simulink model "three_phase_bridge_three_level_ttype_igbt_simple_2th"  (R2026b)
settings: Solver=VariableStepAuto
undefined symbols (not defined in the file): param
libraries: fl_lib x192, nesl_utility x120, igbt_simple_2th_lib x12
(part 1 of 4)
settings Model: Creator=pwr-control  LastModifiedBy=d.bagnara

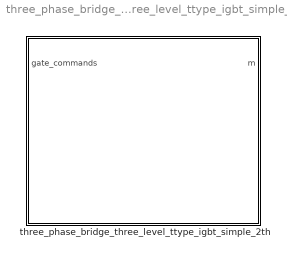
== system three_phase_bridge_three_level_ttype_igbt_simple_2th ==
  three_phase_bridge_three_level_ttype_igbt_simple_2th : Subsystem  mask(three_phase_bridge_three_level_ttype_igbt_simple_2th){vce_sat_m=param.afe.igbt.Vce_sat, rce_on_m=param.afe.igbt.Rce_on*1000, v_gamma_m=param.afe.igbt.Vdon_diode, rd_on_m=param.afe.igbt.Rdon_diode*1e3, Gce_off_m=1e-6, Vth_gate_m=param.afe.igbt.Vth, Vth_gate_hyst_m=0.85, Eon_m=param.afe.igbt.Eon*1000, Eoff_m=param.afe.igbt.Eoff*1000, Err_m=param.afe.igbt.Erec*1000, Ic_ref_m=param.afe.igbt.Ion_sw_losses, Vdc_ref_m=param.afe.igbt.Voff_sw_losses, Vblock_Errf_m=50, time_constant_edge_m=param.glb_time.tc*1e6, time_constant_ploss_m=param.glb_time.tPWM_AFE*5*1e6, Csnubber_m=12e-12, Rsnubber_m=2200, rth_switch_JH_m=param.afe.igbt.Rth_switch_JH, rth_switch_HA_m=param.thermal.Rth_switch_HA, rth_diode_JH_m=param.thermal.Rth_diode_HA, rth_diode_HA_m=param.thermal.Rth_diode_HA, JunctionTermalMass_m=param.afe.igbt.JunctionTermalMass, Tambient_m=param.thermal.Tambient, mass_heatsink_m=param.thermal.weight, specific_heat_m=param.thermal.cp_al}
      mask prompts: vce_sat_m "Collector-emitter on-state voltage (knee) [V]"; rce_on_m "IGBT on-state series resistance (slope) [mOhm]"; v_gamma_m "Diode forward voltage (knee) [V]"; rd_on_m "Diode series resistance (slope) [mOhm]"; Gce_off_m "Off-state conductance [1/Ohm]"; Vth_gate_m "Gate-emitter threshold voltage [V]"; Vth_gate_hyst_m "Half hysteresis band for the switching events [V]"; Eon_m "Turn-on energy at Ic_ref, Vdc_ref [mJ]"; Eoff_m "Turn-off energy at Ic_ref, Vdc_ref [mJ]"; Err_m "Reverse recovery energy at Ic_ref, Vdc_ref [mJ]"; Ic_ref_m "Reference current of the energies [A]"; Vdc_ref_m "Reference voltage of the energies [V]"; Vblock_Errf_m "Blocking detection level for the Err event [V]"; time_constant_edge_m "Sample&hold time constant (<< on-time) [us]"; time_constant_ploss_m "Loss averaging time constant (2-5 x Tsw) [us]"; Csnubber_m "RC snubber capacitance [F]"; Rsnubber_m "RC snubber resistance [Ohm]"; rth_switch_JH_m "Thermal resistance junction-heatsink, transistor die [K/W]"; rth_switch_HA_m "Thermal resistance heatsink-ambient, transistor die [K/W]"; rth_diode_JH_m "Thermal resistance junction-heatsink, diode die [K/W]"; rth_diode_HA_m "Thermal resistance heatsink-ambient, diode die [K/W]"; JunctionTermalMass_m "Junction thermal mass of each die [J/K]"; Tambient_m "Ambient temperature [degC]"; mass_heatsink_m "Heatsink mass seen by each die [kg]"; specific_heat_m "Specific heat of the heatsink [J/(K kg)]"
      mask help: Three-phase bridge, three-level T-type, igbt_simple_2th devices. IGBT cells built on igbt_simple_2th (library/foundation/semiconductors): knee + slope conduction, switching energies scaled from one datasheet point, separate thermal ports for the IGBT and the free-wheeling diode. Each die drives its own junction thermal mass -> Rth JH -> heatsink mass -> Rth HA -> ambient temperature source. Gate command in volts (modulators: +15/-10 V). Bus m per device k: igbt_current, igbt_voltage, igbt_ploss, igbt_JH_temp, igbt_HA_temp, diode_current, diode_ploss, diode_JH_temp, diode_HA_temp (temperatures are differences in K). Default data: Infineon FF450R17ME4 at 125 degC. Ports: gate_commands (bus from the three-level PWM modulators of masked_models/modulators), m (measurement bus), left dc terminals udc(+) / np / udc(-), right ac terminals u / v / w. Device numbering: see three_phase_bridge/README.md.
      mask Help: web('https://github.com/pwr-control/library/blob/dev/library/masked_models/semiconductors_bridges/three_phase_bridge/README.md', '-browser')
      mask DialogControl ParameterGroupVar Prompt: Conduction
      mask DialogControl ParameterGroupVar1 Prompt: Gate
      mask DialogControl ParameterGroupVar2 Prompt: Switching energies
      mask DialogControl ParameterGroupVar3 Prompt: Numerics and snubber
      mask DialogControl ParameterGroupVar4 Prompt: Thermal network
      mask Display:
      | disp(sprintf('three-phase bridge\nT-type 3 levels\nigbt_simple_2th'))
      | port_label('input', 1, 'gate_commands')
      | port_label('output', 1, 'm')
      | port_label('LConn', 1, 'udc(+)')
      | port_label('LConn', 2, 'np')
      | port_label('LConn', 3, 'udc(-)')
      | port_label('RConn', 1, 'u')
      | port_label('RConn', 2, 'v')
      | port_label('RConn', 3, 'w')

== system three_phase_bridge_three_level_ttype_igbt_simple_2th/three_phase_bridge_three_level_ttype_igbt_simple_2th ==
  gate_commands : Inport
  Bus Creator : BusCreator  Inputs=108
  Bus Selector : BusSelector  OutputSignals=gate_cmds_phu.cmd_gate_Q1,gate_cmds_phu.cmd_gate_Q2,gate_cmds_phu.cmd_gate_Q3,gate_cmds_phu.cmd_gate_Q4,gate_cmds_phv.cmd_gate_Q1,gate_cmds_phv.cmd_gate_Q2,gate_cmds_phv.cmd_gate_Q3,gate_cmds_phv.cmd_gate_Q4,gate_cmds_phw.cmd_gate_Q1,gate_cmds_phw.cmd_gate_Q2,gate_cmds_phw.cmd_gate_Q3,gate_cmds_phw.cmd_gate_Q4
  Q1 : Subsystem
  Q10 : Subsystem
  Q11 : Subsystem
  Q12 : Subsystem
  Q2 : Subsystem
  Q3 : Subsystem
  Q4 : Subsystem
  Q5 : Subsystem
  Q6 : Subsystem
  Q7 : Subsystem
  Q8 : Subsystem
  Q9 : Subsystem
  udc(+) : PMIOPort  Side=Left
  np : PMIOPort  Port=2  Side=Left
  udc(-) : PMIOPort  Port=3  Side=Left
  u : PMIOPort  Port=4  Side=Right
  v : PMIOPort  Port=5  Side=Right
  w : PMIOPort  Port=6  Side=Right
  m : Outport
  wires:
  gate_commands/1 -> Bus Selector/1
  Q9/3(p_t) -> Bus Creator/75  "igbt_ploss_Q9"
  Q6/2(v) -> Bus Creator/47  "igbt_voltage_Q6"
  Bus Selector/1 -> Q1/1(g)  "<cmd_gate_Q1>"
  Bus Selector/3 -> Q3/1(g)  "<cmd_gate_Q3>"
  Q3/7(p_d) -> Bus Creator/25  "diode_ploss_Q3"
  Bus Selector/5 -> Q5/1(g)  "<cmd_gate_Q1>"
  Bus Selector/2 -> Q2/1(g)  "<cmd_gate_Q2>"
  Bus Selector/4 -> Q4/1(g)  "<cmd_gate_Q4>"
  Q5/6(i_d) -> Bus Creator/42  "diode_current_Q5"
  Bus Selector/12 -> Q12/1(g)  "<cmd_gate_Q4>"
  Bus Selector/10 -> Q10/1(g)  "<cmd_gate_Q2>"
  Bus Selector/6 -> Q6/1(g)  "<cmd_gate_Q2>"
  Bus Selector/11 -> Q11/1(g)  "<cmd_gate_Q3>"
  Q6/5(dT_HA_t) -> Bus Creator/50  "igbt_HA_temp_Q6"
  Q12/6(i_d) -> Bus Creator/105  "diode_current_Q12"
  Q9/5(dT_HA_t) -> Bus Creator/77  "igbt_HA_temp_Q9"
  Q2/1(i_t) -> Bus Creator/10  "igbt_current_Q2"
  Q11/5(dT_HA_t) -> Bus Creator/95  "igbt_HA_temp_Q11"
  Bus Selector/7 -> Q7/1(g)  "<cmd_gate_Q3>"
  Bus Selector/8 -> Q8/1(g)  "<cmd_gate_Q4>"
  Q6/4(dT_JH_t) -> Bus Creator/49  "igbt_JH_temp_Q6"
  Bus Selector/9 -> Q9/1(g)  "<cmd_gate_Q1>"
  Q5/9(dT_HA_d) -> Bus Creator/45  "diode_HA_temp_Q5"
  Q5/1(i_t) -> Bus Creator/37  "igbt_current_Q5"
  Q1/6(i_d) -> Bus Creator/6  "diode_current_Q1"
  Q9/1(i_t) -> Bus Creator/73  "igbt_current_Q9"
  Q2/7(p_d) -> Bus Creator/16  "diode_ploss_Q2"
  Q9/2(v) -> Bus Creator/74  "igbt_voltage_Q9"
  Q11/4(dT_JH_t) -> Bus Creator/94  "igbt_JH_temp_Q11"
  Q9/4(dT_JH_t) -> Bus Creator/76  "igbt_JH_temp_Q9"
  Q9/6(i_d) -> Bus Creator/78  "diode_current_Q9"
  Q9/7(p_d) -> Bus Creator/79  "diode_ploss_Q9"
  Q9/8(dT_JH_d) -> Bus Creator/80  "diode_JH_temp_Q9"
  Q9/9(dT_HA_d) -> Bus Creator/81  "diode_HA_temp_Q9"
  Q1/4(dT_JH_t) -> Bus Creator/4  "igbt_JH_temp_Q1"
  Q1/1(i_t) -> Bus Creator/1  "igbt_current_Q1"
  Q4/8(dT_JH_d) -> Bus Creator/35  "diode_JH_temp_Q4"
  Q5/4(dT_JH_t) -> Bus Creator/40  "igbt_JH_temp_Q5"
  Q1/9(dT_HA_d) -> Bus Creator/9  "diode_HA_temp_Q1"
  Q1/5(dT_HA_t) -> Bus Creator/5  "igbt_HA_temp_Q1"
  Q1/2(v) -> Bus Creator/2  "igbt_voltage_Q1"
  Q1/3(p_t) -> Bus Creator/3  "igbt_ploss_Q1"
  Q5/5(dT_HA_t) -> Bus Creator/41  "igbt_HA_temp_Q5"
  Q10/9(dT_HA_d) -> Bus Creator/90  "diode_HA_temp_Q10"
  Q1/7(p_d) -> Bus Creator/7  "diode_ploss_Q1"
  Q1/8(dT_JH_d) -> Bus Creator/8  "diode_JH_temp_Q1"
  Q2/2(v) -> Bus Creator/11  "igbt_voltage_Q2"
  Q2/3(p_t) -> Bus Creator/12  "igbt_ploss_Q2"
  Q6/9(dT_HA_d) -> Bus Creator/54  "diode_HA_temp_Q6"
  Q5/8(dT_JH_d) -> Bus Creator/44  "diode_JH_temp_Q5"
  Q2/4(dT_JH_t) -> Bus Creator/13  "igbt_JH_temp_Q2"
  Q2/5(dT_HA_t) -> Bus Creator/14  "igbt_HA_temp_Q2"
  Q12/3(p_t) -> Bus Creator/102  "igbt_ploss_Q12"
  Q2/6(i_d) -> Bus Creator/15  "diode_current_Q2"
  Q5/3(p_t) -> Bus Creator/39  "igbt_ploss_Q5"
  Q2/8(dT_JH_d) -> Bus Creator/17  "diode_JH_temp_Q2"
  Q2/9(dT_HA_d) -> Bus Creator/18  "diode_HA_temp_Q2"
  Q6/1(i_t) -> Bus Creator/46  "igbt_current_Q6"
  Q6/7(p_d) -> Bus Creator/52  "diode_ploss_Q6"
  Q5/2(v) -> Bus Creator/38  "igbt_voltage_Q5"
  Q5/7(p_d) -> Bus Creator/43  "diode_ploss_Q5"
  Q6/3(p_t) -> Bus Creator/48  "igbt_ploss_Q6"
  Q6/6(i_d) -> Bus Creator/51  "diode_current_Q6"
  Q6/8(dT_JH_d) -> Bus Creator/53  "diode_JH_temp_Q6"
  Q10/1(i_t) -> Bus Creator/82  "igbt_current_Q10"
  Q10/2(v) -> Bus Creator/83  "igbt_voltage_Q10"
  Q10/3(p_t) -> Bus Creator/84  "igbt_ploss_Q10"
  Q10/4(dT_JH_t) -> Bus Creator/85  "igbt_JH_temp_Q10"
  Q10/5(dT_HA_t) -> Bus Creator/86  "igbt_HA_temp_Q10"
  Q10/6(i_d) -> Bus Creator/87  "diode_current_Q10"
  Q10/7(p_d) -> Bus Creator/88  "diode_ploss_Q10"
  Q10/8(dT_JH_d) -> Bus Creator/89  "diode_JH_temp_Q10"
  Q12/1(i_t) -> Bus Creator/100  "igbt_current_Q12"
  Q12/2(v) -> Bus Creator/101  "igbt_voltage_Q12"
  Q11/2(v) -> Bus Creator/92  "igbt_voltage_Q11"
  Q12/4(dT_JH_t) -> Bus Creator/103  "igbt_JH_temp_Q12"
  Q12/5(dT_HA_t) -> Bus Creator/104  "igbt_HA_temp_Q12"
  Q12/7(p_d) -> Bus Creator/106  "diode_ploss_Q12"
  Q4/3(p_t) -> Bus Creator/30  "igbt_ploss_Q4"
  Q12/8(dT_JH_d) -> Bus Creator/107  "diode_JH_temp_Q12"
  Q12/9(dT_HA_d) -> Bus Creator/108  "diode_HA_temp_Q12"
  Q3/1(i_t) -> Bus Creator/19  "igbt_current_Q3"
  Q3/2(v) -> Bus Creator/20  "igbt_voltage_Q3"
  Q3/3(p_t) -> Bus Creator/21  "igbt_ploss_Q3"
  Q3/4(dT_JH_t) -> Bus Creator/22  "igbt_JH_temp_Q3"
  Q3/5(dT_HA_t) -> Bus Creator/23  "igbt_HA_temp_Q3"
  Q3/6(i_d) -> Bus Creator/24  "diode_current_Q3"
  Q3/8(dT_JH_d) -> Bus Creator/26  "diode_JH_temp_Q3"
  Q3/9(dT_HA_d) -> Bus Creator/27  "diode_HA_temp_Q3"
  Q4/1(i_t) -> Bus Creator/28  "igbt_current_Q4"
  Q4/2(v) -> Bus Creator/29  "igbt_voltage_Q4"
  Q4/4(dT_JH_t) -> Bus Creator/31  "igbt_JH_temp_Q4"
  Q4/5(dT_HA_t) -> Bus Creator/32  "igbt_HA_temp_Q4"
  Q11/9(dT_HA_d) -> Bus Creator/99  "diode_HA_temp_Q11"
  Q4/6(i_d) -> Bus Creator/33  "diode_current_Q4"
  Q4/7(p_d) -> Bus Creator/34  "diode_ploss_Q4"
  Q4/9(dT_HA_d) -> Bus Creator/36  "diode_HA_temp_Q4"
  Q7/1(i_t) -> Bus Creator/55  "igbt_current_Q7"
  Q7/2(v) -> Bus Creator/56  "igbt_voltage_Q7"
  Q7/3(p_t) -> Bus Creator/57  "igbt_ploss_Q7"
  Q7/4(dT_JH_t) -> Bus Creator/58  "igbt_JH_temp_Q7"
  Q7/5(dT_HA_t) -> Bus Creator/59  "igbt_HA_temp_Q7"
  Q7/6(i_d) -> Bus Creator/60  "diode_current_Q7"
  Q7/7(p_d) -> Bus Creator/61  "diode_ploss_Q7"
  Q7/8(dT_JH_d) -> Bus Creator/62  "diode_JH_temp_Q7"
  Q7/9(dT_HA_d) -> Bus Creator/63  "diode_HA_temp_Q7"
  Q8/1(i_t) -> Bus Creator/64  "igbt_current_Q8"
  Q8/2(v) -> Bus Creator/65  "igbt_voltage_Q8"
  Q8/3(p_t) -> Bus Creator/66  "igbt_ploss_Q8"
  Q8/4(dT_JH_t) -> Bus Creator/67  "igbt_JH_temp_Q8"
  Q8/5(dT_HA_t) -> Bus Creator/68  "igbt_HA_temp_Q8"
  Q8/6(i_d) -> Bus Creator/69  "diode_current_Q8"
  Q8/7(p_d) -> Bus Creator/70  "diode_ploss_Q8"
  Q8/8(dT_JH_d) -> Bus Creator/71  "diode_JH_temp_Q8"
  Q8/9(dT_HA_d) -> Bus Creator/72  "diode_HA_temp_Q8"
  Q11/1(i_t) -> Bus Creator/91  "igbt_current_Q11"
  Q11/3(p_t) -> Bus Creator/93  "igbt_ploss_Q11"
  Q11/6(i_d) -> Bus Creator/96  "diode_current_Q11"
  Q11/7(p_d) -> Bus Creator/97  "diode_ploss_Q11"
  Q11/8(dT_JH_d) -> Bus Creator/98  "diode_JH_temp_Q11"
  Bus Creator/1 -> m/1  "m"
  connections:
  udc(+)/RConn1 -- Q1/LConn1 -- Q5/LConn1 -- Q9/LConn1
  Q1/RConn1 -- Q3/LConn1 -- Q4/LConn1 -- u/RConn1
  np/RConn1 -- Q2/LConn1 -- Q6/LConn1 -- Q10/LConn1
  Q12/RConn1 -- Q8/RConn1 -- Q4/RConn1 -- udc(-)/RConn1
  Q9/RConn1 -- Q12/LConn1 -- w/RConn1 -- Q11/LConn1
  Q2/RConn1 -- Q3/RConn1
  Q5/RConn1 -- Q8/LConn1 -- Q7/LConn1 -- v/RConn1
  Q6/RConn1 -- Q7/RConn1
  Q10/RConn1 -- Q11/RConn1

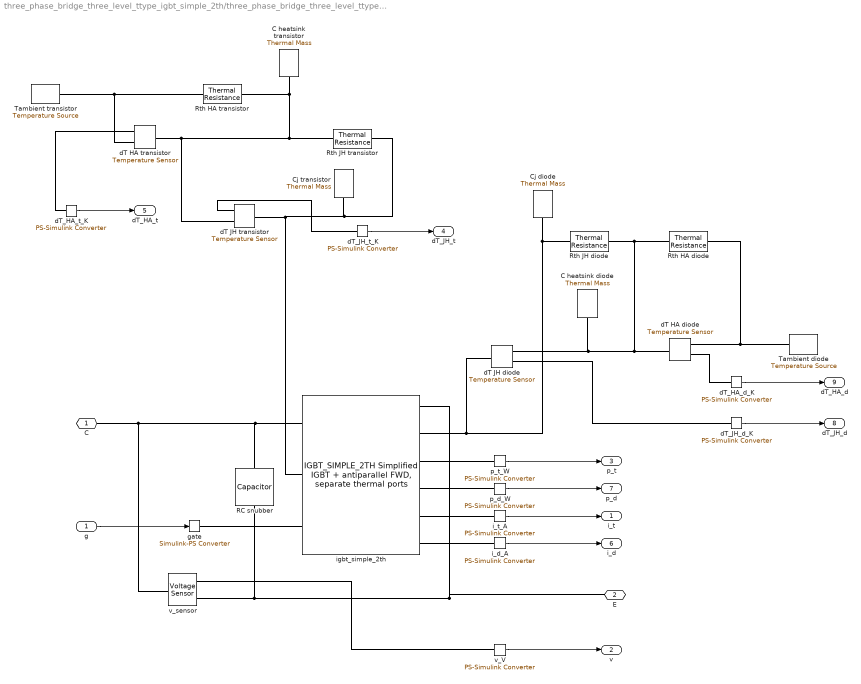
== system three_phase_bridge_three_level_ttype_igbt_simple_2th/three_phase_bridge_three_level_ttype_igbt_simple_2th/Q1 ==
  g : Inport
  C heatsink diode : fl_lib/Thermal/Thermal Elements/Thermal Mass  mass_type=foundation.enum.constant_variable.constant  mass=mass_heatsink_m kg  sp_heat=specific_heat_m J/(K*kg)  mass_min=1e-6 kg  num_ports=foundation.enum.numPorts2.one  m_specify=off  m_priority=High  m=1 kg  m_nominal_specify=off  m_nominal_value=1  m_nominal_unit=kg  T_specify=on  T_priority=High  T=Tambient_m degC  T_nominal_specify=off  T_nominal_value=1  T_nominal_unit=K  Q_specify=off  Q_priority=High  Q=0 W  Q_nominal_specify=off  Q_nominal_value=1  Q_nominal_unit=W
  C heatsink transistor : fl_lib/Thermal/Thermal Elements/Thermal Mass  mass_type=foundation.enum.constant_variable.constant  mass=mass_heatsink_m kg  sp_heat=specific_heat_m J/(K*kg)  mass_min=1e-6 kg  num_ports=foundation.enum.numPorts2.one  m_specify=off  m_priority=High  m=1 kg  m_nominal_specify=off  m_nominal_value=1  m_nominal_unit=kg  T_specify=on  T_priority=High  T=Tambient_m degC  T_nominal_specify=off  T_nominal_value=1  T_nominal_unit=K  Q_specify=off  Q_priority=High  Q=0 W  Q_nominal_specify=off  Q_nominal_value=1  Q_nominal_unit=W
  Cj diode : fl_lib/Thermal/Thermal Elements/Thermal Mass  mass_type=foundation.enum.constant_variable.constant  mass=JunctionTermalMass_m/specific_heat_m kg  sp_heat=specific_heat_m J/(K*kg)  mass_min=1e-6 kg  num_ports=foundation.enum.numPorts2.one  m_specify=off  m_priority=High  m=1 kg  m_nominal_specify=off  m_nominal_value=1  m_nominal_unit=kg  T_specify=on  T_priority=High  T=Tambient_m degC  T_nominal_specify=off  T_nominal_value=1  T_nominal_unit=K  Q_specify=off  Q_priority=High  Q=0 W  Q_nominal_specify=off  Q_nominal_value=1  Q_nominal_unit=W
  Cj transistor : fl_lib/Thermal/Thermal Elements/Thermal Mass  mass_type=foundation.enum.constant_variable.constant  mass=JunctionTermalMass_m/specific_heat_m kg  sp_heat=specific_heat_m J/(K*kg)  mass_min=1e-6 kg  num_ports=foundation.enum.numPorts2.one  m_specify=off  m_priority=High  m=1 kg  m_nominal_specify=off  m_nominal_value=1  m_nominal_unit=kg  T_specify=on  T_priority=High  T=Tambient_m degC  T_nominal_specify=off  T_nominal_value=1  T_nominal_unit=K  Q_specify=off  Q_priority=High  Q=0 W  Q_nominal_specify=off  Q_nominal_value=1  Q_nominal_unit=W
  RC snubber : fl_lib/Electrical/Electrical Elements/Capacitor  c=Csnubber_m F  r=Rsnubber_m Ohm  g=0 1/Ohm  i_specify=off  i_priority=None  i=0 A  i_nominal_specify=off  i_nominal_value=1  i_nominal_unit=A  v_specify=off  v_priority=None  v=0 V  v_nominal_specify=off  v_nominal_value=1  v_nominal_unit=V  vc_specify=off  vc_priority=High  vc=0 V  vc_nominal_specify=off  vc_nominal_value=1  vc_nominal_unit=V
  Rth HA diode : fl_lib/Thermal/Thermal Elements/Thermal Resistance  resistance=rth_diode_HA_m K/W  T_specify=off  T_priority=High  T=0 deltadegC  T_nominal_specify=off  T_nominal_value=1  T_nominal_unit=K  Q_specify=off  Q_priority=None  Q=0 W  Q_nominal_specify=off  Q_nominal_value=1  Q_nominal_unit=W
  Rth HA transistor : fl_lib/Thermal/Thermal Elements/Thermal Resistance  resistance=rth_switch_HA_m K/W  T_specify=off  T_priority=High  T=0 deltadegC  T_nominal_specify=off  T_nominal_value=1  T_nominal_unit=K  Q_specify=off  Q_priority=None  Q=0 W  Q_nominal_specify=off  Q_nominal_value=1  Q_nominal_unit=W
  Rth JH diode : fl_lib/Thermal/Thermal Elements/Thermal Resistance  resistance=rth_diode_JH_m K/W  T_specify=off  T_priority=High  T=0 deltadegC  T_nominal_specify=off  T_nominal_value=1  T_nominal_unit=K  Q_specify=off  Q_priority=None  Q=0 W  Q_nominal_specify=off  Q_nominal_value=1  Q_nominal_unit=W
  Rth JH transistor : fl_lib/Thermal/Thermal Elements/Thermal Resistance  resistance=rth_switch_JH_m K/W  T_specify=off  T_priority=High  T=0 deltadegC  T_nominal_specify=off  T_nominal_value=1  T_nominal_unit=K  Q_specify=off  Q_priority=None  Q=0 W  Q_nominal_specify=off  Q_nominal_value=1  Q_nominal_unit=W
  Tambient diode : fl_lib/Thermal/Thermal Sources/Temperature Source  temperature=Tambient_m degC
  Tambient transistor : fl_lib/Thermal/Thermal Sources/Temperature Source  temperature=Tambient_m degC
  dT HA diode : fl_lib/Thermal/Thermal Sensors/Temperature Sensor  temperature_measure=foundation.enum.MeasurementReference.difference
  dT HA transistor : fl_lib/Thermal/Thermal Sensors/Temperature Sensor  temperature_measure=foundation.enum.MeasurementReference.difference
  dT JH diode : fl_lib/Thermal/Thermal Sensors/Temperature Sensor  temperature_measure=foundation.enum.MeasurementReference.difference
  dT JH transistor : fl_lib/Thermal/Thermal Sensors/Temperature Sensor  temperature_measure=foundation.enum.MeasurementReference.difference
  dT_HA_d_K : nesl_utility/PS-Simulink Converter  PhysicalDomain=network_engine_domain  SubClassName=ps_output  LeftPortType=input  RightPortType=output  PseudoPeriodic=off  Frequencies=[]  VectorFormat=1-D array  Unit=K  AffineConversion=off
  dT_HA_t_K : nesl_utility/PS-Simulink Converter  PhysicalDomain=network_engine_domain  SubClassName=ps_output  LeftPortType=input  RightPortType=output  PseudoPeriodic=off  Frequencies=[]  VectorFormat=1-D array  Unit=K  AffineConversion=off
  dT_JH_d_K : nesl_utility/PS-Simulink Converter  PhysicalDomain=network_engine_domain  SubClassName=ps_output  LeftPortType=input  RightPortType=output  PseudoPeriodic=off  Frequencies=[]  VectorFormat=1-D array  Unit=K  AffineConversion=off
  dT_JH_t_K : nesl_utility/PS-Simulink Converter  PhysicalDomain=network_engine_domain  SubClassName=ps_output  LeftPortType=input  RightPortType=output  PseudoPeriodic=off  Frequencies=[]  VectorFormat=1-D array  Unit=K  AffineConversion=off
  gate : nesl_utility/Simulink-PS Converter  PhysicalDomain=network_engine_domain  SubClassName=ps_input  LeftPortType=input  RightPortType=output  PseudoPeriodic=off  Frequencies=[]  NoiseDistribution=none  NoiseParameters=[]  Unit=V  AffineConversion=off  FilteringAndDerivatives=provide  SimscapeFilterOrder=1  InputFilterTimeConstant=0.001  UdotUserProvided=0
  i_d_A : nesl_utility/PS-Simulink Converter  PhysicalDomain=network_engine_domain  SubClassName=ps_output  LeftPortType=input  RightPortType=output  PseudoPeriodic=off  Frequencies=[]  VectorFormat=1-D array  Unit=A  AffineConversion=off
  i_t_A : nesl_utility/PS-Simulink Converter  PhysicalDomain=network_engine_domain  SubClassName=ps_output  LeftPortType=input  RightPortType=output  PseudoPeriodic=off  Frequencies=[]  VectorFormat=1-D array  Unit=A  AffineConversion=off
  igbt_simple_2th : igbt_simple_2th_lib/IGBT_SIMPLE_2TH Simplified IGBT + antiparallel FWD, separate thermal ports  Vce_sat=vce_sat_m V  Vf=v_gamma_m V  Vth=Vth_gate_m V  Vhyst=Vth_gate_hyst_m V  Eon_ref=Eon_m mJ  Eoff_ref=Eoff_m mJ  Err_ref=Err_m mJ  Ic_ref=Ic_ref_m A  Vdc_ref=Vdc_ref_m V  V_rr_th=Vblock_Errf_m V  Ron=rce_on_m mOhm  Rd=rd_on_m mOhm  Goff=Gce_off_m 1/Ohm  tau_s=time_constant_edge_m us  tau_p=time_constant_ploss_m us  i_specify=off  i_priority=None  i=0 A  i_nominal_specify=off  i_nominal_value=1  i_nominal_unit=A  v_specify=off  v_priority=None  v=0 V  v_nominal_specify=off  v_nominal_value=1  v_nominal_unit=V  i_t_specify=off  i_t_priority=None  i_t=0 A  i_t_nominal_specify=off  i_t_nominal_value=1  i_t_nominal_unit=A  i_d_specify=off  i_d_priority=None  i_d=0 A  i_d_nominal_specify=off  i_d_nominal_value=1  i_d_nominal_unit=A  i_h_specify=off  i_h_priority=None  i_h=0 A  i_h_nominal_specify=off  i_h_nominal_value=1  i_h_nominal_unit=A  i_dh_specify=off  i_dh_priority=None  i_dh=0 A  i_dh_nominal_specify=off  i_dh_nominal_value=1  i_dh_nominal_unit=A  v_h_specify=off  v_h_priority=None  v_h=0 V  v_h_nominal_specify=off  v_h_nominal_value=1  v_h_nominal_unit=V  E_lpt_specify=off  E_lpt_priority=None  E_lpt=0 J  E_lpt_nominal_specify=off  E_lpt_nominal_value=1  E_lpt_nominal_unit=J  E_lpd_specify=off  E_lpd_priority=None  E_lpd=0 J  E_lpd_nominal_specify=off  E_lpd_nominal_value=1  E_lpd_nominal_unit=J  Qt_specify=off  Qt_priority=None  Qt=0 W  Qt_nominal_specify=off  Qt_nominal_value=1  Qt_nominal_unit=W  Qd_specify=off  Qd_priority=None  Qd=0 W  Qd_nominal_specify=off  Qd_nominal_value=1  Qd_nominal_unit=W  E_t_specify=off  E_t_priority=None  E_t=0 J  E_d_specify=off  E_d_priority=None  E_d=0 J
  p_d_W : nesl_utility/PS-Simulink Converter  PhysicalDomain=network_engine_domain  SubClassName=ps_output  LeftPortType=input  RightPortType=output  PseudoPeriodic=off  Frequencies=[]  VectorFormat=1-D array  Unit=W  AffineConversion=off
  p_t_W : nesl_utility/PS-Simulink Converter  PhysicalDomain=network_engine_domain  SubClassName=ps_output  LeftPortType=input  RightPortType=output  PseudoPeriodic=off  Frequencies=[]  VectorFormat=1-D array  Unit=W  AffineConversion=off
  v_V : nesl_utility/PS-Simulink Converter  PhysicalDomain=network_engine_domain  SubClassName=ps_output  LeftPortType=input  RightPortType=output  PseudoPeriodic=off  Frequencies=[]  VectorFormat=1-D array  Unit=V  AffineConversion=off
  v_sensor : fl_lib/Electrical/Electrical Sensors/Voltage Sensor
  C : PMIOPort  Side=Left
  E : PMIOPort  Port=2  Side=Right
  i_t : Outport
  v : Outport  Port=2
  p_t : Outport  Port=3
  dT_JH_t : Outport  Port=4
  dT_HA_t : Outport  Port=5
  i_d : Outport  Port=6
  p_d : Outport  Port=7
  dT_JH_d : Outport  Port=8
  dT_HA_d : Outport  Port=9
  wires:
  v_V/1 -> v/1
  g/1 -> gate/1
  dT_HA_t_K/1 -> dT_HA_t/1
  dT_JH_d_K/1 -> dT_JH_d/1
  dT_JH_t_K/1 -> dT_JH_t/1
  p_t_W/1 -> p_t/1
  p_d_W/1 -> p_d/1
  i_t_A/1 -> i_t/1
  i_d_A/1 -> i_d/1
  dT_HA_d_K/1 -> dT_HA_d/1
  connections:
  Tambient transistor/LConn1 -- dT HA transistor/RConn1 -- Rth HA transistor/RConn1
  dT HA transistor/LConn1 -- Rth HA transistor/LConn1 -- C heatsink transistor/LConn1 -- Rth JH transistor/RConn1 -- dT JH transistor/RConn1
  dT JH transistor/LConn1 -- igbt_simple_2th/LConn2 -- Cj transistor/LConn1 -- Rth JH transistor/LConn1
  dT HA transistor/RConn2 -- dT_HA_t_K/LConn1
  C/RConn1 -- igbt_simple_2th/LConn1 -- RC snubber/LConn1 -- v_sensor/LConn1
  dT JH diode/RConn2 -- dT_JH_d_K/LConn1
  igbt_simple_2th/RConn5 -- i_t_A/LConn1
  igbt_simple_2th/RConn4 -- p_d_W/LConn1
  dT JH transistor/RConn2 -- dT_JH_t_K/LConn1
  gate/RConn1 -- igbt_simple_2th/LConn3
  v_sensor/RConn1 -- v_V/LConn1
  v_sensor/RConn2 -- igbt_simple_2th/RConn1 -- E/RConn1 -- RC snubber/RConn1
  igbt_simple_2th/RConn2 -- Rth JH diode/LConn1 -- Cj diode/LConn1 -- dT JH diode/LConn1
  dT HA diode/RConn2 -- dT_HA_d_K/LConn1
  igbt_simple_2th/RConn3 -- p_t_W/LConn1
  dT JH diode/RConn1 -- Rth JH diode/RConn1 -- Rth HA diode/LConn1 -- dT HA diode/LConn1 -- C heatsink diode/LConn1
  igbt_simple_2th/RConn6 -- i_d_A/LConn1
  dT HA diode/RConn1 -- Rth HA diode/RConn1 -- Tambient diode/LConn1

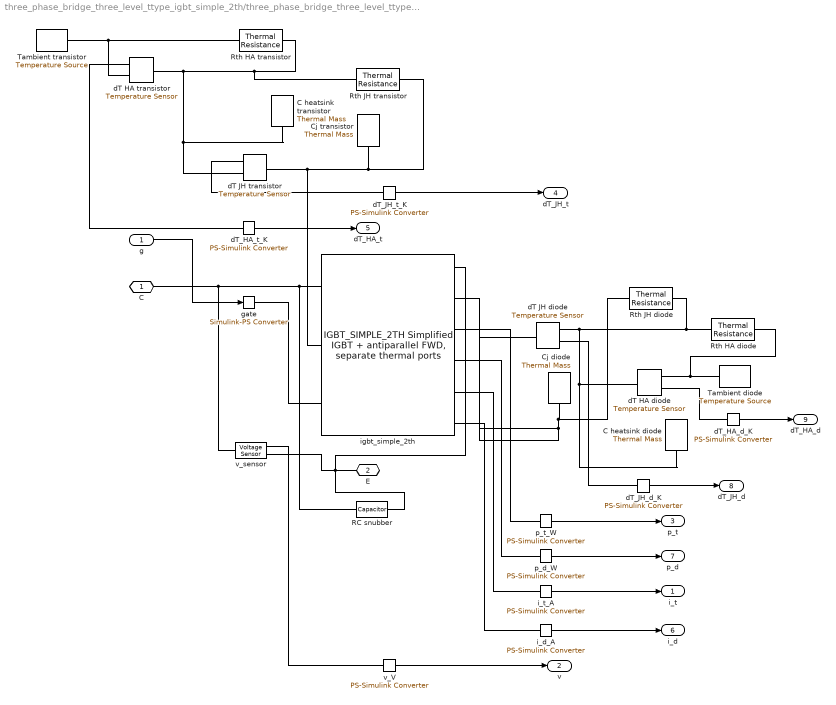
== system three_phase_bridge_three_level_ttype_igbt_simple_2th/three_phase_bridge_three_level_ttype_igbt_simple_2th/Q10 ==
  g : Inport
  C heatsink diode : fl_lib/Thermal/Thermal Elements/Thermal Mass  mass_type=foundation.enum.constant_variable.constant  mass=mass_heatsink_m kg  sp_heat=specific_heat_m J/(K*kg)  mass_min=1e-6 kg  num_ports=foundation.enum.numPorts2.one  m_specify=off  m_priority=High  m=1 kg  m_nominal_specify=off  m_nominal_value=1  m_nominal_unit=kg  T_specify=on  T_priority=High  T=Tambient_m degC  T_nominal_specify=off  T_nominal_value=1  T_nominal_unit=K  Q_specify=off  Q_priority=High  Q=0 W  Q_nominal_specify=off  Q_nominal_value=1  Q_nominal_unit=W
  C heatsink transistor : fl_lib/Thermal/Thermal Elements/Thermal Mass  mass_type=foundation.enum.constant_variable.constant  mass=mass_heatsink_m kg  sp_heat=specific_heat_m J/(K*kg)  mass_min=1e-6 kg  num_ports=foundation.enum.numPorts2.one  m_specify=off  m_priority=High  m=1 kg  m_nominal_specify=off  m_nominal_value=1  m_nominal_unit=kg  T_specify=on  T_priority=High  T=Tambient_m degC  T_nominal_specify=off  T_nominal_value=1  T_nominal_unit=K  Q_specify=off  Q_priority=High  Q=0 W  Q_nominal_specify=off  Q_nominal_value=1  Q_nominal_unit=W
  Cj diode : fl_lib/Thermal/Thermal Elements/Thermal Mass  mass_type=foundation.enum.constant_variable.constant  mass=JunctionTermalMass_m/specific_heat_m kg  sp_heat=specific_heat_m J/(K*kg)  mass_min=1e-6 kg  num_ports=foundation.enum.numPorts2.one  m_specify=off  m_priority=High  m=1 kg  m_nominal_specify=off  m_nominal_value=1  m_nominal_unit=kg  T_specify=on  T_priority=High  T=Tambient_m degC  T_nominal_specify=off  T_nominal_value=1  T_nominal_unit=K  Q_specify=off  Q_priority=High  Q=0 W  Q_nominal_specify=off  Q_nominal_value=1  Q_nominal_unit=W
  Cj transistor : fl_lib/Thermal/Thermal Elements/Thermal Mass  mass_type=foundation.enum.constant_variable.constant  mass=JunctionTermalMass_m/specific_heat_m kg  sp_heat=specific_heat_m J/(K*kg)  mass_min=1e-6 kg  num_ports=foundation.enum.numPorts2.one  m_specify=off  m_priority=High  m=1 kg  m_nominal_specify=off  m_nominal_value=1  m_nominal_unit=kg  T_specify=on  T_priority=High  T=Tambient_m degC  T_nominal_specify=off  T_nominal_value=1  T_nominal_unit=K  Q_specify=off  Q_priority=High  Q=0 W  Q_nominal_specify=off  Q_nominal_value=1  Q_nominal_unit=W
  RC snubber : fl_lib/Electrical/Electrical Elements/Capacitor  c=Csnubber_m F  r=Rsnubber_m Ohm  g=0 1/Ohm  i_specify=off  i_priority=None  i=0 A  i_nominal_specify=off  i_nominal_value=1  i_nominal_unit=A  v_specify=off  v_priority=None  v=0 V  v_nominal_specify=off  v_nominal_value=1  v_nominal_unit=V  vc_specify=off  vc_priority=High  vc=0 V  vc_nominal_specify=off  vc_nominal_value=1  vc_nominal_unit=V
  Rth HA diode : fl_lib/Thermal/Thermal Elements/Thermal Resistance  resistance=rth_diode_HA_m K/W  T_specify=off  T_priority=High  T=0 deltadegC  T_nominal_specify=off  T_nominal_value=1  T_nominal_unit=K  Q_specify=off  Q_priority=None  Q=0 W  Q_nominal_specify=off  Q_nominal_value=1  Q_nominal_unit=W
  Rth HA transistor : fl_lib/Thermal/Thermal Elements/Thermal Resistance  resistance=rth_switch_HA_m K/W  T_specify=off  T_priority=High  T=0 deltadegC  T_nominal_specify=off  T_nominal_value=1  T_nominal_unit=K  Q_specify=off  Q_priority=None  Q=0 W  Q_nominal_specify=off  Q_nominal_value=1  Q_nominal_unit=W
  Rth JH diode : fl_lib/Thermal/Thermal Elements/Thermal Resistance  resistance=rth_diode_JH_m K/W  T_specify=off  T_priority=High  T=0 deltadegC  T_nominal_specify=off  T_nominal_value=1  T_nominal_unit=K  Q_specify=off  Q_priority=None  Q=0 W  Q_nominal_specify=off  Q_nominal_value=1  Q_nominal_unit=W
  Rth JH transistor : fl_lib/Thermal/Thermal Elements/Thermal Resistance  resistance=rth_switch_JH_m K/W  T_specify=off  T_priority=High  T=0 deltadegC  T_nominal_specify=off  T_nominal_value=1  T_nominal_unit=K  Q_specify=off  Q_priority=None  Q=0 W  Q_nominal_specify=off  Q_nominal_value=1  Q_nominal_unit=W
  Tambient diode : fl_lib/Thermal/Thermal Sources/Temperature Source  temperature=Tambient_m degC
  Tambient transistor : fl_lib/Thermal/Thermal Sources/Temperature Source  temperature=Tambient_m degC
  dT HA diode : fl_lib/Thermal/Thermal Sensors/Temperature Sensor  temperature_measure=foundation.enum.MeasurementReference.difference
  dT HA transistor : fl_lib/Thermal/Thermal Sensors/Temperature Sensor  temperature_measure=foundation.enum.MeasurementReference.difference
  dT JH diode : fl_lib/Thermal/Thermal Sensors/Temperature Sensor  temperature_measure=foundation.enum.MeasurementReference.difference
  dT JH transistor : fl_lib/Thermal/Thermal Sensors/Temperature Sensor  temperature_measure=foundation.enum.MeasurementReference.difference
  dT_HA_d_K : nesl_utility/PS-Simulink Converter  PhysicalDomain=network_engine_domain  SubClassName=ps_output  LeftPortType=input  RightPortType=output  PseudoPeriodic=off  Frequencies=[]  VectorFormat=1-D array  Unit=K  AffineConversion=off
  dT_HA_t_K : nesl_utility/PS-Simulink Converter  PhysicalDomain=network_engine_domain  SubClassName=ps_output  LeftPortType=input  RightPortType=output  PseudoPeriodic=off  Frequencies=[]  VectorFormat=1-D array  Unit=K  AffineConversion=off
  dT_JH_d_K : nesl_utility/PS-Simulink Converter  PhysicalDomain=network_engine_domain  SubClassName=ps_output  LeftPortType=input  RightPortType=output  PseudoPeriodic=off  Frequencies=[]  VectorFormat=1-D array  Unit=K  AffineConversion=off
  dT_JH_t_K : nesl_utility/PS-Simulink Converter  PhysicalDomain=network_engine_domain  SubClassName=ps_output  LeftPortType=input  RightPortType=output  PseudoPeriodic=off  Frequencies=[]  VectorFormat=1-D array  Unit=K  AffineConversion=off
  gate : nesl_utility/Simulink-PS Converter  PhysicalDomain=network_engine_domain  SubClassName=ps_input  LeftPortType=input  RightPortType=output  PseudoPeriodic=off  Frequencies=[]  NoiseDistribution=none  NoiseParameters=[]  Unit=V  AffineConversion=off  FilteringAndDerivatives=provide  SimscapeFilterOrder=1  InputFilterTimeConstant=0.001  UdotUserProvided=0
  i_d_A : nesl_utility/PS-Simulink Converter  PhysicalDomain=network_engine_domain  SubClassName=ps_output  LeftPortType=input  RightPortType=output  PseudoPeriodic=off  Frequencies=[]  VectorFormat=1-D array  Unit=A  AffineConversion=off
  i_t_A : nesl_utility/PS-Simulink Converter  PhysicalDomain=network_engine_domain  SubClassName=ps_output  LeftPortType=input  RightPortType=output  PseudoPeriodic=off  Frequencies=[]  VectorFormat=1-D array  Unit=A  AffineConversion=off
  igbt_simple_2th : igbt_simple_2th_lib/IGBT_SIMPLE_2TH Simplified IGBT + antiparallel FWD, separate thermal ports  Vce_sat=vce_sat_m V  Vf=v_gamma_m V  Vth=Vth_gate_m V  Vhyst=Vth_gate_hyst_m V  Eon_ref=Eon_m mJ  Eoff_ref=Eoff_m mJ  Err_ref=Err_m mJ  Ic_ref=Ic_ref_m A  Vdc_ref=Vdc_ref_m V  V_rr_th=Vblock_Errf_m V  Ron=rce_on_m mOhm  Rd=rd_on_m mOhm  Goff=Gce_off_m 1/Ohm  tau_s=time_constant_edge_m us  tau_p=time_constant_ploss_m us  i_specify=off  i_priority=None  i=0 A  i_nominal_specify=off  i_nominal_value=1  i_nominal_unit=A  v_specify=off  v_priority=None  v=0 V  v_nominal_specify=off  v_nominal_value=1  v_nominal_unit=V  i_t_specify=off  i_t_priority=None  i_t=0 A  i_t_nominal_specify=off  i_t_nominal_value=1  i_t_nominal_unit=A  i_d_specify=off  i_d_priority=None  i_d=0 A  i_d_nominal_specify=off  i_d_nominal_value=1  i_d_nominal_unit=A  i_h_specify=off  i_h_priority=None  i_h=0 A  i_h_nominal_specify=off  i_h_nominal_value=1  i_h_nominal_unit=A  i_dh_specify=off  i_dh_priority=None  i_dh=0 A  i_dh_nominal_specify=off  i_dh_nominal_value=1  i_dh_nominal_unit=A  v_h_specify=off  v_h_priority=None  v_h=0 V  v_h_nominal_specify=off  v_h_nominal_value=1  v_h_nominal_unit=V  E_lpt_specify=off  E_lpt_priority=None  E_lpt=0 J  E_lpt_nominal_specify=off  E_lpt_nominal_value=1  E_lpt_nominal_unit=J  E_lpd_specify=off  E_lpd_priority=None  E_lpd=0 J  E_lpd_nominal_specify=off  E_lpd_nominal_value=1  E_lpd_nominal_unit=J  Qt_specify=off  Qt_priority=None  Qt=0 W  Qt_nominal_specify=off  Qt_nominal_value=1  Qt_nominal_unit=W  Qd_specify=off  Qd_priority=None  Qd=0 W  Qd_nominal_specify=off  Qd_nominal_value=1  Qd_nominal_unit=W  E_t_specify=off  E_t_priority=None  E_t=0 J  E_d_specify=off  E_d_priority=None  E_d=0 J
  p_d_W : nesl_utility/PS-Simulink Converter  PhysicalDomain=network_engine_domain  SubClassName=ps_output  LeftPortType=input  RightPortType=output  PseudoPeriodic=off  Frequencies=[]  VectorFormat=1-D array  Unit=W  AffineConversion=off
  p_t_W : nesl_utility/PS-Simulink Converter  PhysicalDomain=network_engine_domain  SubClassName=ps_output  LeftPortType=input  RightPortType=output  PseudoPeriodic=off  Frequencies=[]  VectorFormat=1-D array  Unit=W  AffineConversion=off
  v_V : nesl_utility/PS-Simulink Converter  PhysicalDomain=network_engine_domain  SubClassName=ps_output  LeftPortType=input  RightPortType=output  PseudoPeriodic=off  Frequencies=[]  VectorFormat=1-D array  Unit=V  AffineConversion=off
  v_sensor : fl_lib/Electrical/Electrical Sensors/Voltage Sensor
  C : PMIOPort  Side=Left
  E : PMIOPort  Port=2  Side=Right
  i_t : Outport
  v : Outport  Port=2
  p_t : Outport  Port=3
  dT_JH_t : Outport  Port=4
  dT_HA_t : Outport  Port=5
  i_d : Outport  Port=6
  p_d : Outport  Port=7
  dT_JH_d : Outport  Port=8
  dT_HA_d : Outport  Port=9
  wires:
  v_V/1 -> v/1
  dT_HA_t_K/1 -> dT_HA_t/1
  g/1 -> gate/1
  dT_JH_t_K/1 -> dT_JH_t/1
  p_d_W/1 -> p_d/1
  dT_JH_d_K/1 -> dT_JH_d/1
  i_t_A/1 -> i_t/1
  dT_HA_d_K/1 -> dT_HA_d/1
  p_t_W/1 -> p_t/1
  i_d_A/1 -> i_d/1
  connections:
  gate/RConn1 -- igbt_simple_2th/LConn3
  dT HA transistor/RConn2 -- dT_HA_t_K/LConn1
  Tambient transistor/LConn1 -- Rth HA transistor/RConn1 -- dT HA transistor/RConn1
  dT HA transistor/LConn1 -- C heatsink transistor/LConn1 -- dT JH transistor/RConn1 -- Rth HA transistor/LConn1 -- Rth JH transistor/RConn1
  dT JH transistor/RConn2 -- dT_JH_t_K/LConn1
  C/RConn1 -- igbt_simple_2th/LConn1 -- RC snubber/LConn1 -- v_sensor/LConn1
  igbt_simple_2th/RConn6 -- i_d_A/LConn1
  dT JH transistor/LConn1 -- Cj transistor/LConn1 -- Rth JH transistor/LConn1 -- igbt_simple_2th/LConn2
  v_sensor/RConn1 -- v_V/LConn1
  v_sensor/RConn2 -- E/RConn1 -- igbt_simple_2th/RConn1 -- RC snubber/RConn1
  igbt_simple_2th/RConn2 -- Cj diode/LConn1 -- Rth JH diode/LConn1 -- dT JH diode/LConn1
  igbt_simple_2th/RConn3 -- p_t_W/LConn1
  igbt_simple_2th/RConn4 -- p_d_W/LConn1
  igbt_simple_2th/RConn5 -- i_t_A/LConn1
  dT JH diode/RConn1 -- C heatsink diode/LConn1 -- dT HA diode/LConn1 -- Rth HA diode/LConn1 -- Rth JH diode/RConn1
  dT JH diode/RConn2 -- dT_JH_d_K/LConn1
  dT HA diode/RConn1 -- Rth HA diode/RConn1 -- Tambient diode/LConn1
  dT HA diode/RConn2 -- dT_HA_d_K/LConn1

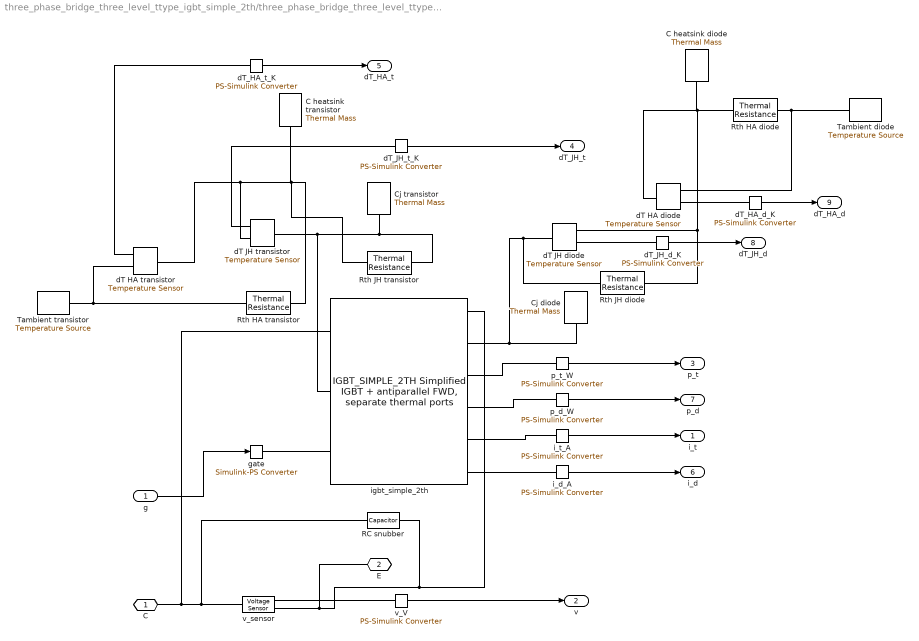
== system three_phase_bridge_three_level_ttype_igbt_simple_2th/three_phase_bridge_three_level_ttype_igbt_simple_2th/Q11 ==
  g : Inport
  C heatsink diode : fl_lib/Thermal/Thermal Elements/Thermal Mass  mass_type=foundation.enum.constant_variable.constant  mass=mass_heatsink_m kg  sp_heat=specific_heat_m J/(K*kg)  mass_min=1e-6 kg  num_ports=foundation.enum.numPorts2.one  m_specify=off  m_priority=High  m=1 kg  m_nominal_specify=off  m_nominal_value=1  m_nominal_unit=kg  T_specify=on  T_priority=High  T=Tambient_m degC  T_nominal_specify=off  T_nominal_value=1  T_nominal_unit=K  Q_specify=off  Q_priority=High  Q=0 W  Q_nominal_specify=off  Q_nominal_value=1  Q_nominal_unit=W
  C heatsink transistor : fl_lib/Thermal/Thermal Elements/Thermal Mass  mass_type=foundation.enum.constant_variable.constant  mass=mass_heatsink_m kg  sp_heat=specific_heat_m J/(K*kg)  mass_min=1e-6 kg  num_ports=foundation.enum.numPorts2.one  m_specify=off  m_priority=High  m=1 kg  m_nominal_specify=off  m_nominal_value=1  m_nominal_unit=kg  T_specify=on  T_priority=High  T=Tambient_m degC  T_nominal_specify=off  T_nominal_value=1  T_nominal_unit=K  Q_specify=off  Q_priority=High  Q=0 W  Q_nominal_specify=off  Q_nominal_value=1  Q_nominal_unit=W
  Cj diode : fl_lib/Thermal/Thermal Elements/Thermal Mass  mass_type=foundation.enum.constant_variable.constant  mass=JunctionTermalMass_m/specific_heat_m kg  sp_heat=specific_heat_m J/(K*kg)  mass_min=1e-6 kg  num_ports=foundation.enum.numPorts2.one  m_specify=off  m_priority=High  m=1 kg  m_nominal_specify=off  m_nominal_value=1  m_nominal_unit=kg  T_specify=on  T_priority=High  T=Tambient_m degC  T_nominal_specify=off  T_nominal_value=1  T_nominal_unit=K  Q_specify=off  Q_priority=High  Q=0 W  Q_nominal_specify=off  Q_nominal_value=1  Q_nominal_unit=W
  Cj transistor : fl_lib/Thermal/Thermal Elements/Thermal Mass  mass_type=foundation.enum.constant_variable.constant  mass=JunctionTermalMass_m/specific_heat_m kg  sp_heat=specific_heat_m J/(K*kg)  mass_min=1e-6 kg  num_ports=foundation.enum.numPorts2.one  m_specify=off  m_priority=High  m=1 kg  m_nominal_specify=off  m_nominal_value=1  m_nominal_unit=kg  T_specify=on  T_priority=High  T=Tambient_m degC  T_nominal_specify=off  T_nominal_value=1  T_nominal_unit=K  Q_specify=off  Q_priority=High  Q=0 W  Q_nominal_specify=off  Q_nominal_value=1  Q_nominal_unit=W
  RC snubber : fl_lib/Electrical/Electrical Elements/Capacitor  c=Csnubber_m F  r=Rsnubber_m Ohm  g=0 1/Ohm  i_specify=off  i_priority=None  i=0 A  i_nominal_specify=off  i_nominal_value=1  i_nominal_unit=A  v_specify=off  v_priority=None  v=0 V  v_nominal_specify=off  v_nominal_value=1  v_nominal_unit=V  vc_specify=off  vc_priority=High  vc=0 V  vc_nominal_specify=off  vc_nominal_value=1  vc_nominal_unit=V
  Rth HA diode : fl_lib/Thermal/Thermal Elements/Thermal Resistance  resistance=rth_diode_HA_m K/W  T_specify=off  T_priority=High  T=0 deltadegC  T_nominal_specify=off  T_nominal_value=1  T_nominal_unit=K  Q_specify=off  Q_priority=None  Q=0 W  Q_nominal_specify=off  Q_nominal_value=1  Q_nominal_unit=W
  Rth HA transistor : fl_lib/Thermal/Thermal Elements/Thermal Resistance  resistance=rth_switch_HA_m K/W  T_specify=off  T_priority=High  T=0 deltadegC  T_nominal_specify=off  T_nominal_value=1  T_nominal_unit=K  Q_specify=off  Q_priority=None  Q=0 W  Q_nominal_specify=off  Q_nominal_value=1  Q_nominal_unit=W
  Rth JH diode : fl_lib/Thermal/Thermal Elements/Thermal Resistance  resistance=rth_diode_JH_m K/W  T_specify=off  T_priority=High  T=0 deltadegC  T_nominal_specify=off  T_nominal_value=1  T_nominal_unit=K  Q_specify=off  Q_priority=None  Q=0 W  Q_nominal_specify=off  Q_nominal_value=1  Q_nominal_unit=W
  Rth JH transistor : fl_lib/Thermal/Thermal Elements/Thermal Resistance  resistance=rth_switch_JH_m K/W  T_specify=off  T_priority=High  T=0 deltadegC  T_nominal_specify=off  T_nominal_value=1  T_nominal_unit=K  Q_specify=off  Q_priority=None  Q=0 W  Q_nominal_specify=off  Q_nominal_value=1  Q_nominal_unit=W
  Tambient diode : fl_lib/Thermal/Thermal Sources/Temperature Source  temperature=Tambient_m degC
  Tambient transistor : fl_lib/Thermal/Thermal Sources/Temperature Source  temperature=Tambient_m degC
  dT HA diode : fl_lib/Thermal/Thermal Sensors/Temperature Sensor  temperature_measure=foundation.enum.MeasurementReference.difference
  dT HA transistor : fl_lib/Thermal/Thermal Sensors/Temperature Sensor  temperature_measure=foundation.enum.MeasurementReference.difference
  dT JH diode : fl_lib/Thermal/Thermal Sensors/Temperature Sensor  temperature_measure=foundation.enum.MeasurementReference.difference
  dT JH transistor : fl_lib/Thermal/Thermal Sensors/Temperature Sensor  temperature_measure=foundation.enum.MeasurementReference.difference
  dT_HA_d_K : nesl_utility/PS-Simulink Converter  PhysicalDomain=network_engine_domain  SubClassName=ps_output  LeftPortType=input  RightPortType=output  PseudoPeriodic=off  Frequencies=[]  VectorFormat=1-D array  Unit=K  AffineConversion=off
  dT_HA_t_K : nesl_utility/PS-Simulink Converter  PhysicalDomain=network_engine_domain  SubClassName=ps_output  LeftPortType=input  RightPortType=output  PseudoPeriodic=off  Frequencies=[]  VectorFormat=1-D array  Unit=K  AffineConversion=off
  dT_JH_d_K : nesl_utility/PS-Simulink Converter  PhysicalDomain=network_engine_domain  SubClassName=ps_output  LeftPortType=input  RightPortType=output  PseudoPeriodic=off  Frequencies=[]  VectorFormat=1-D array  Unit=K  AffineConversion=off
  dT_JH_t_K : nesl_utility/PS-Simulink Converter  PhysicalDomain=network_engine_domain  SubClassName=ps_output  LeftPortType=input  RightPortType=output  PseudoPeriodic=off  Frequencies=[]  VectorFormat=1-D array  Unit=K  AffineConversion=off
  gate : nesl_utility/Simulink-PS Converter  PhysicalDomain=network_engine_domain  SubClassName=ps_input  LeftPortType=input  RightPortType=output  PseudoPeriodic=off  Frequencies=[]  NoiseDistribution=none  NoiseParameters=[]  Unit=V  AffineConversion=off  FilteringAndDerivatives=provide  SimscapeFilterOrder=1  InputFilterTimeConstant=0.001  UdotUserProvided=0
  i_d_A : nesl_utility/PS-Simulink Converter  PhysicalDomain=network_engine_domain  SubClassName=ps_output  LeftPortType=input  RightPortType=output  PseudoPeriodic=off  Frequencies=[]  VectorFormat=1-D array  Unit=A  AffineConversion=off
  i_t_A : nesl_utility/PS-Simulink Converter  PhysicalDomain=network_engine_domain  SubClassName=ps_output  LeftPortType=input  RightPortType=output  PseudoPeriodic=off  Frequencies=[]  VectorFormat=1-D array  Unit=A  AffineConversion=off
  igbt_simple_2th : igbt_simple_2th_lib/IGBT_SIMPLE_2TH Simplified IGBT + antiparallel FWD, separate thermal ports  Vce_sat=vce_sat_m V  Vf=v_gamma_m V  Vth=Vth_gate_m V  Vhyst=Vth_gate_hyst_m V  Eon_ref=Eon_m mJ  Eoff_ref=Eoff_m mJ  Err_ref=Err_m mJ  Ic_ref=Ic_ref_m A  Vdc_ref=Vdc_ref_m V  V_rr_th=Vblock_Errf_m V  Ron=rce_on_m mOhm  Rd=rd_on_m mOhm  Goff=Gce_off_m 1/Ohm  tau_s=time_constant_edge_m us  tau_p=time_constant_ploss_m us  i_specify=off  i_priority=None  i=0 A  i_nominal_specify=off  i_nominal_value=1  i_nominal_unit=A  v_specify=off  v_priority=None  v=0 V  v_nominal_specify=off  v_nominal_value=1  v_nominal_unit=V  i_t_specify=off  i_t_priority=None  i_t=0 A  i_t_nominal_specify=off  i_t_nominal_value=1  i_t_nominal_unit=A  i_d_specify=off  i_d_priority=None  i_d=0 A  i_d_nominal_specify=off  i_d_nominal_value=1  i_d_nominal_unit=A  i_h_specify=off  i_h_priority=None  i_h=0 A  i_h_nominal_specify=off  i_h_nominal_value=1  i_h_nominal_unit=A  i_dh_specify=off  i_dh_priority=None  i_dh=0 A  i_dh_nominal_specify=off  i_dh_nominal_value=1  i_dh_nominal_unit=A  v_h_specify=off  v_h_priority=None  v_h=0 V  v_h_nominal_specify=off  v_h_nominal_value=1  v_h_nominal_unit=V  E_lpt_specify=off  E_lpt_priority=None  E_lpt=0 J  E_lpt_nominal_specify=off  E_lpt_nominal_value=1  E_lpt_nominal_unit=J  E_lpd_specify=off  E_lpd_priority=None  E_lpd=0 J  E_lpd_nominal_specify=off  E_lpd_nominal_value=1  E_lpd_nominal_unit=J  Qt_specify=off  Qt_priority=None  Qt=0 W  Qt_nominal_specify=off  Qt_nominal_value=1  Qt_nominal_unit=W  Qd_specify=off  Qd_priority=None  Qd=0 W  Qd_nominal_specify=off  Qd_nominal_value=1  Qd_nominal_unit=W  E_t_specify=off  E_t_priority=None  E_t=0 J  E_d_specify=off  E_d_priority=None  E_d=0 J
  p_d_W : nesl_utility/PS-Simulink Converter  PhysicalDomain=network_engine_domain  SubClassName=ps_output  LeftPortType=input  RightPortType=output  PseudoPeriodic=off  Frequencies=[]  VectorFormat=1-D array  Unit=W  AffineConversion=off
  p_t_W : nesl_utility/PS-Simulink Converter  PhysicalDomain=network_engine_domain  SubClassName=ps_output  LeftPortType=input  RightPortType=output  PseudoPeriodic=off  Frequencies=[]  VectorFormat=1-D array  Unit=W  AffineConversion=off
  v_V : nesl_utility/PS-Simulink Converter  PhysicalDomain=network_engine_domain  SubClassName=ps_output  LeftPortType=input  RightPortType=output  PseudoPeriodic=off  Frequencies=[]  VectorFormat=1-D array  Unit=V  AffineConversion=off
  v_sensor : fl_lib/Electrical/Electrical Sensors/Voltage Sensor
  C : PMIOPort  Side=Left
  E : PMIOPort  Port=2  Side=Right
  i_t : Outport
  v : Outport  Port=2
  p_t : Outport  Port=3
  dT_JH_t : Outport  Port=4
  dT_HA_t : Outport  Port=5
  i_d : Outport  Port=6
  p_d : Outport  Port=7
  dT_JH_d : Outport  Port=8
  dT_HA_d : Outport  Port=9
  wires:
  g/1 -> gate/1
  dT_JH_d_K/1 -> dT_JH_d/1
  p_d_W/1 -> p_d/1
  dT_HA_t_K/1 -> dT_HA_t/1
  dT_JH_t_K/1 -> dT_JH_t/1
  i_d_A/1 -> i_d/1
  v_V/1 -> v/1
  p_t_W/1 -> p_t/1
  i_t_A/1 -> i_t/1
  dT_HA_d_K/1 -> dT_HA_d/1
  connections:
  Tambient transistor/LConn1 -- Rth HA transistor/RConn1 -- dT HA transistor/RConn1
  C/RConn1 -- v_sensor/LConn1 -- RC snubber/LConn1 -- igbt_simple_2th/LConn1
  dT HA transistor/RConn2 -- dT_HA_t_K/LConn1
  dT HA transistor/LConn1 -- C heatsink transistor/LConn1 -- Rth JH transistor/RConn1 -- Rth HA transistor/LConn1 -- dT JH transistor/RConn1
  dT JH transistor/RConn2 -- dT_JH_t_K/LConn1
  dT JH transistor/LConn1 -- Cj transistor/LConn1 -- Rth JH transistor/LConn1 -- igbt_simple_2th/LConn2
  gate/RConn1 -- igbt_simple_2th/LConn3
  v_sensor/RConn1 -- v_V/LConn1
  v_sensor/RConn2 -- RC snubber/RConn1 -- igbt_simple_2th/RConn1 -- E/RConn1
  igbt_simple_2th/RConn3 -- p_t_W/LConn1
  igbt_simple_2th/RConn2 -- dT JH diode/LConn1 -- Rth JH diode/LConn1 -- Cj diode/LConn1
  igbt_simple_2th/RConn4 -- p_d_W/LConn1
  igbt_simple_2th/RConn5 -- i_t_A/LConn1
  igbt_simple_2th/RConn6 -- i_d_A/LConn1
  dT JH diode/RConn1 -- dT HA diode/LConn1 -- C heatsink diode/LConn1 -- Rth HA diode/LConn1 -- Rth JH diode/RConn1
  dT JH diode/RConn2 -- dT_JH_d_K/LConn1
  dT HA diode/RConn1 -- Rth HA diode/RConn1 -- Tambient diode/LConn1
  dT HA diode/RConn2 -- dT_HA_d_K/LConn1
